simulink model "IEEE33BusTestSystem_Instantaneous"  (R2019a)
settings: Solver=FixedStepAuto  StartTime=0.0  StopTime=0.2  FixedStep=50e-6  RelTol=1e-3
libraries: powerlib x141, powerlib_meascontrol x2
(part 3 of 3)

== system IEEE33BusTestSystem_Instantaneous/Bus_7 ==
  Bus Load 7 : powerlib/Elements/Three-Phase Series RLC Load  LConnTagsString=A|B|C  Configuration=Y (grounded)  NominalVoltage=(12660)*0.946243  Vabc=[1e3 1e3 1e3]  Vabcp=[1e3 1e3 1e3]  NominalFrequency=50  UnbalancedPower=off  ActivePower=200e3  InductivePower=100e3  CapacitivePower=0  Pabc=[10e3 9e3 11e3]  QLabc=[100 90 110]  QCabc=[100 90 110]  Pabcp=[10e3 9e3 11e3]  QLabcp=[100 90 110]  QCabcp=[100 90 110]  Measurements=None  LoadType=constant PQ
      settings: SourceProductName=Simscape Electrical
  Bus_7 : powerlib/Measurements/Three-Phase V-I Measurement  VoltageMeasurement=phase-to-phase  SetLabelV=off  LabelV=Vabc  Vpu=off  VpuLL=off  CurrentMeasurement=yes  SetLabelI=off  LabelI=Iabc  Ipu=off  Pbase=100e6  Vbase=500e3  OutputType=Complex  PhasorSimulation=off  PSBequivalent=0
      settings: SourceProductName=Simscape Electrical
  CB3-2 : powerlib/Elements/Three-Phase Breaker  InitialState=open  SwitchA=on  SwitchB=on  SwitchC=on  SwitchTimes="[1/60  5/60]"  External=on  BreakerResistance=0.01  SnubberResistance=1e6  SnubberCapacitance=inf  Measurements=None
      settings: SourceProductName=Simscape Electrical
  VI Recorder10 : Subsystem
  InPhaseA : PMIOPort  Side=Left
  InPhaseB : PMIOPort  Port=2  Side=Left
  InPhaseC : PMIOPort  Port=3  Side=Left
  OutPhaseA : PMIOPort  Port=4  Side=Right
  OutPhaseB : PMIOPort  Port=5  Side=Right
  OutPhaseC : PMIOPort  Port=6  Side=Right
  wires:
  Bus_7/2 -> VI Recorder10/2(Irec)
  Bus_7/1 -> VI Recorder10/1(Vrec)
  [CB7to8] -> CB3-2/1
  connections:
  Bus_7/RConn1 -- CB3-2/LConn1 -- Bus Load 7/LConn1
  CB3-2/RConn3 -- OutPhaseC/RConn1
  Bus Load 7/LConn2 -- CB3-2/LConn2 -- Bus_7/RConn2
  CB3-2/LConn3 -- Bus Load 7/LConn3 -- Bus_7/RConn3
  CB3-2/RConn1 -- OutPhaseA/RConn1
  CB3-2/RConn2 -- OutPhaseB/RConn1
  InPhaseA/RConn1 -- Bus_7/LConn1
  InPhaseB/RConn1 -- Bus_7/LConn2
  InPhaseC/RConn1 -- Bus_7/LConn3

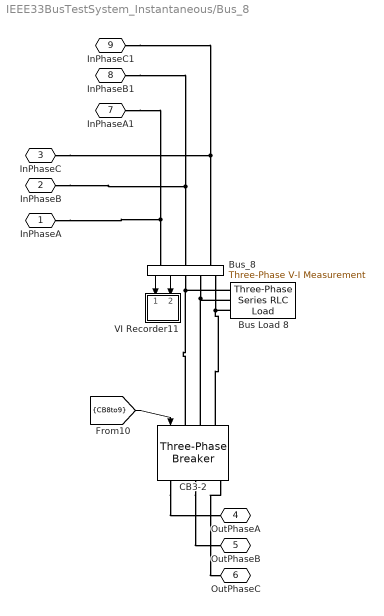
== system IEEE33BusTestSystem_Instantaneous/Bus_8 ==
  Bus Load 8 : powerlib/Elements/Three-Phase Series RLC Load  LConnTagsString=A|B|C  Configuration=Y (grounded)  NominalVoltage=(12660)*0.941407  Vabc=[1e3 1e3 1e3]  Vabcp=[1e3 1e3 1e3]  NominalFrequency=50  UnbalancedPower=off  ActivePower=200e3  InductivePower=100e3  CapacitivePower=0  Pabc=[10e3 9e3 11e3]  QLabc=[100 90 110]  QCabc=[100 90 110]  Pabcp=[10e3 9e3 11e3]  QLabcp=[100 90 110]  QCabcp=[100 90 110]  Measurements=None  LoadType=constant PQ
      settings: SourceProductName=Simscape Electrical
  Bus_8 : powerlib/Measurements/Three-Phase V-I Measurement  VoltageMeasurement=phase-to-phase  SetLabelV=off  LabelV=Vabc  Vpu=off  VpuLL=off  CurrentMeasurement=yes  SetLabelI=off  LabelI=Iabc  Ipu=off  Pbase=100e6  Vbase=500e3  OutputType=Complex  PhasorSimulation=off  PSBequivalent=0
      settings: SourceProductName=Simscape Electrical
  CB3-2 : powerlib/Elements/Three-Phase Breaker  InitialState=open  SwitchA=on  SwitchB=on  SwitchC=on  SwitchTimes="[1/60  5/60]"  External=on  BreakerResistance=0.01  SnubberResistance=1e6  SnubberCapacitance=inf  Measurements=None
      settings: SourceProductName=Simscape Electrical
  VI Recorder11 : Subsystem
  InPhaseA : PMIOPort  Side=Left
  InPhaseB : PMIOPort  Port=2  Side=Left
  InPhaseC : PMIOPort  Port=3  Side=Left
  OutPhaseA : PMIOPort  Port=4  Side=Right
  OutPhaseB : PMIOPort  Port=5  Side=Right
  OutPhaseC : PMIOPort  Port=6  Side=Right
  InPhaseA1 : PMIOPort  Port=7  Side=Left
  InPhaseB1 : PMIOPort  Port=8  Side=Left
  InPhaseC1 : PMIOPort  Port=9  Side=Left
  wires:
  Bus_8/2 -> VI Recorder11/2(Irec)
  Bus_8/1 -> VI Recorder11/1(Vrec)
  [CB8to9] -> CB3-2/1
  connections:
  Bus Load 8/LConn1 -- CB3-2/LConn1 -- Bus_8/RConn1
  CB3-2/RConn3 -- OutPhaseC/RConn1
  Bus Load 8/LConn2 -- CB3-2/LConn2 -- Bus_8/RConn2
  Bus_8/RConn3 -- CB3-2/LConn3 -- Bus Load 8/LConn3
  CB3-2/RConn1 -- OutPhaseA/RConn1
  CB3-2/RConn2 -- OutPhaseB/RConn1
  InPhaseA1/RConn1 -- InPhaseA/RConn1 -- Bus_8/LConn1
  InPhaseB1/RConn1 -- InPhaseB/RConn1 -- Bus_8/LConn2
  InPhaseC1/RConn1 -- InPhaseC/RConn1 -- Bus_8/LConn3

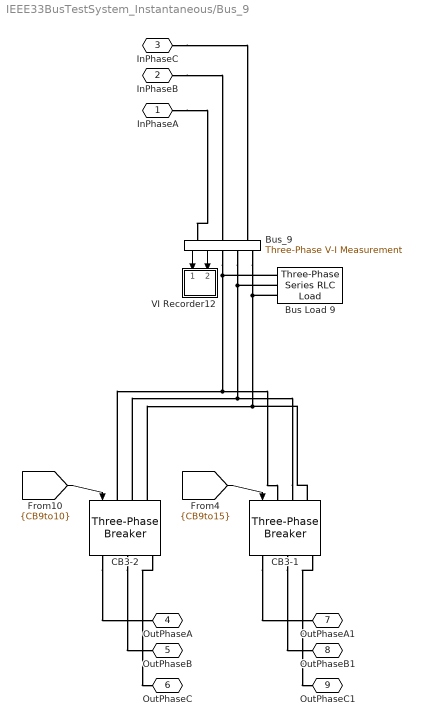
== system IEEE33BusTestSystem_Instantaneous/Bus_9 ==
  Bus Load 9 : powerlib/Elements/Three-Phase Series RLC Load  LConnTagsString=A|B|C  Configuration=Y (grounded)  NominalVoltage=(12660)*0.935148  Vabc=[1e3 1e3 1e3]  Vabcp=[1e3 1e3 1e3]  NominalFrequency=50  UnbalancedPower=off  ActivePower=60e3  InductivePower=20e3  CapacitivePower=0  Pabc=[10e3 9e3 11e3]  QLabc=[100 90 110]  QCabc=[100 90 110]  Pabcp=[10e3 9e3 11e3]  QLabcp=[100 90 110]  QCabcp=[100 90 110]  Measurements=None  LoadType=constant PQ
      settings: SourceProductName=Simscape Electrical
  Bus_9 : powerlib/Measurements/Three-Phase V-I Measurement  VoltageMeasurement=phase-to-phase  SetLabelV=off  LabelV=Vabc  Vpu=off  VpuLL=off  CurrentMeasurement=yes  SetLabelI=off  LabelI=Iabc  Ipu=off  Pbase=100e6  Vbase=500e3  OutputType=Complex  PhasorSimulation=off  PSBequivalent=0
      settings: SourceProductName=Simscape Electrical
  CB3-1 : powerlib/Elements/Three-Phase Breaker  InitialState=open  SwitchA=on  SwitchB=on  SwitchC=on  SwitchTimes="[1/60  5/60]"  External=on  BreakerResistance=0.01  SnubberResistance=1e6  SnubberCapacitance=inf  Measurements=None
      settings: SourceProductName=Simscape Electrical
  CB3-2 : powerlib/Elements/Three-Phase Breaker  InitialState=open  SwitchA=on  SwitchB=on  SwitchC=on  SwitchTimes="[1/60  5/60]"  External=on  BreakerResistance=0.01  SnubberResistance=1e6  SnubberCapacitance=inf  Measurements=None
      settings: SourceProductName=Simscape Electrical
  VI Recorder12 : Subsystem
  InPhaseA : PMIOPort  Side=Left
  InPhaseB : PMIOPort  Port=2  Side=Left
  InPhaseC : PMIOPort  Port=3  Side=Left
  OutPhaseA : PMIOPort  Port=4  Side=Right
  OutPhaseB : PMIOPort  Port=5  Side=Right
  OutPhaseC : PMIOPort  Port=6  Side=Right
  OutPhaseA1 : PMIOPort  Port=7  Side=Right
  OutPhaseB1 : PMIOPort  Port=8  Side=Right
  OutPhaseC1 : PMIOPort  Port=9  Side=Right
  wires:
  Bus_9/2 -> VI Recorder12/2(Irec)
  Bus_9/1 -> VI Recorder12/1(Vrec)
  [CB9to10] -> CB3-2/1
  [CB9to15] -> CB3-1/1
  connections:
  CB3-1/LConn1 -- Bus Load 9/LConn1 -- Bus_9/RConn1 -- CB3-2/LConn1
  CB3-2/RConn3 -- OutPhaseC/RConn1
  CB3-1/LConn2 -- Bus_9/RConn2 -- Bus Load 9/LConn2 -- CB3-2/LConn2
  Bus Load 9/LConn3 -- Bus_9/RConn3 -- CB3-1/LConn3 -- CB3-2/LConn3
  CB3-2/RConn1 -- OutPhaseA/RConn1
  CB3-2/RConn2 -- OutPhaseB/RConn1
  InPhaseA/RConn1 -- Bus_9/LConn1
  InPhaseB/RConn1 -- Bus_9/LConn2
  InPhaseC/RConn1 -- Bus_9/LConn3
  CB3-1/RConn2 -- OutPhaseB1/RConn1
  CB3-1/RConn3 -- OutPhaseC1/RConn1
  CB3-1/RConn1 -- OutPhaseA1/RConn1

== system IEEE33BusTestSystem_Instantaneous/Bus_10/VI Recorder13 ==
  Vrec : Inport
  Irec : Inport  Port=2
  tag scope: I9to10=global, V9to10=global
  wires:
  Vrec/1 -> [V9to10]
  Irec/1 -> [I9to10]

== system IEEE33BusTestSystem_Instantaneous/Bus_11/VI Recorder14 ==
  Vrec : Inport
  Irec : Inport  Port=2
  tag scope: I10to11=global, V10to11=global
  wires:
  Vrec/1 -> [V10to11]
  Irec/1 -> [I10to11]

== system IEEE33BusTestSystem_Instantaneous/Bus_12/VI Recorder15 ==
  Vrec : Inport
  Irec : Inport  Port=2
  tag scope: I11to12=global, V11to12=global
  wires:
  Vrec/1 -> [V11to12]
  Irec/1 -> [I11to12]

== system IEEE33BusTestSystem_Instantaneous/Bus_13/VI Recorder16 ==
  Vrec : Inport
  Irec : Inport  Port=2
  tag scope: I12to13=global, V12to13=global
  wires:
  Vrec/1 -> [V12to13]
  Irec/1 -> [I12to13]

== system IEEE33BusTestSystem_Instantaneous/Bus_14/VI Recorder17 ==
  Vrec : Inport
  Irec : Inport  Port=2
  tag scope: I13to14=global, V13to14=global
  wires:
  Vrec/1 -> [V13to14]
  Irec/1 -> [I13to14]

== system IEEE33BusTestSystem_Instantaneous/Bus_15/VI Recorder18 ==
  Vrec : Inport
  Irec : Inport  Port=2
  tag scope: I14to15=global, V14to15=global
  wires:
  Vrec/1 -> [V14to15]
  Irec/1 -> [I14to15]

== system IEEE33BusTestSystem_Instantaneous/Bus_16/VI Recorder19 ==
  Vrec : Inport
  Irec : Inport  Port=2
  tag scope: I15to16=global, V15to16=global
  wires:
  Vrec/1 -> [V15to16]
  Irec/1 -> [I15to16]

== system IEEE33BusTestSystem_Instantaneous/Bus_17/VI Recorder20 ==
  Vrec : Inport
  Irec : Inport  Port=2
  tag scope: I16to17=global, V16to17=global
  wires:
  Vrec/1 -> [V16to17]
  Irec/1 -> [I16to17]

== system IEEE33BusTestSystem_Instantaneous/Bus_18/VI Recorder21 ==
  Vrec : Inport
  Irec : Inport  Port=2
  tag scope: I17to18=global, V17to18=global
  wires:
  Vrec/1 -> [V17to18]
  Irec/1 -> [I17to18]

== system IEEE33BusTestSystem_Instantaneous/Bus_19/VI Recorder ==
  Vrec : Inport
  Irec : Inport  Port=2
  tag scope: I2to19=global, V2to19=global
  wires:
  Vrec/1 -> [V2to19]
  Irec/1 -> [I2to19]

== system IEEE33BusTestSystem_Instantaneous/Bus_2/VI Recorder5 ==
  Vrec : Inport
  Irec : Inport  Port=2
  tag scope: I1to2=global, V1to2=global
  wires:
  Vrec/1 -> [V1to2]
  Irec/1 -> [I1to2]

== system IEEE33BusTestSystem_Instantaneous/Bus_20/VI Recorder1 ==
  Vrec : Inport
  Irec : Inport  Port=2
  tag scope: I19to20=global, V19to20=global
  wires:
  Vrec/1 -> [V19to20]
  Irec/1 -> [I19to20]

== system IEEE33BusTestSystem_Instantaneous/Bus_21/VI Recorder2 ==
  Vrec : Inport
  Irec : Inport  Port=2
  tag scope: I20to21=global, V20to21=global
  wires:
  Vrec/1 -> [V20to21]
  Irec/1 -> [I20to21]

== system IEEE33BusTestSystem_Instantaneous/Bus_22/VI Recorder3 ==
  Vrec : Inport
  Irec : Inport  Port=2
  tag scope: I21to22=global, V21to22=global
  wires:
  Vrec/1 -> [V21to22]
  Irec/1 -> [I21to22]

== system IEEE33BusTestSystem_Instantaneous/Bus_23/VI Recorder32 ==
  Vrec : Inport
  Irec : Inport  Port=2
  tag scope: I3to23=global, V3to23=global
  wires:
  Vrec/1 -> [V3to23]
  Irec/1 -> [I3to23]

== system IEEE33BusTestSystem_Instantaneous/Bus_24/VI Recorder31 ==
  Vrec : Inport
  Irec : Inport  Port=2
  tag scope: I23to24=global, V23to24=global
  wires:
  Vrec/1 -> [V23to24]
  Irec/1 -> [I23to24]

== system IEEE33BusTestSystem_Instantaneous/Bus_25/VI Recorder30 ==
  Vrec : Inport
  Irec : Inport  Port=2
  tag scope: I24to25=global, V24to25=global
  wires:
  Vrec/1 -> [V24to25]
  Irec/1 -> [I24to25]

== system IEEE33BusTestSystem_Instantaneous/Bus_26/VI Recorder22 ==
  Vrec : Inport
  Irec : Inport  Port=2
  tag scope: I6to26=global, V6to26=global
  wires:
  Vrec/1 -> [V6to26]
  Irec/1 -> [I6to26]

== system IEEE33BusTestSystem_Instantaneous/Bus_27/VI Recorder23 ==
  Vrec : Inport
  Irec : Inport  Port=2
  tag scope: I26to27=global, V26to27=global
  wires:
  Vrec/1 -> [V26to27]
  Irec/1 -> [I26to27]

== system IEEE33BusTestSystem_Instantaneous/Bus_28/VI Recorder24 ==
  Vrec : Inport
  Irec : Inport  Port=2
  tag scope: I27to28=global, V27to28=global
  wires:
  Vrec/1 -> [V27to28]
  Irec/1 -> [I27to28]

== system IEEE33BusTestSystem_Instantaneous/Bus_29/VI Recorder25 ==
  Vrec : Inport
  Irec : Inport  Port=2
  tag scope: I28to29=global, V28to29=global
  wires:
  Vrec/1 -> [V28to29]
  Irec/1 -> [I28to29]

== system IEEE33BusTestSystem_Instantaneous/Bus_3/VI Recorder6 ==
  Vrec : Inport
  Irec : Inport  Port=2
  tag scope: I2to3=global, V2to3=global
  wires:
  Vrec/1 -> [V2to3]
  Irec/1 -> [I2to3]

== system IEEE33BusTestSystem_Instantaneous/Bus_30/VI Recorder26 ==
  Vrec : Inport
  Irec : Inport  Port=2
  tag scope: I29to30=global, V29to30=global
  wires:
  Vrec/1 -> [V29to30]
  Irec/1 -> [I29to30]

== system IEEE33BusTestSystem_Instantaneous/Bus_31/VI Recorder27 ==
  Vrec : Inport
  Irec : Inport  Port=2
  tag scope: I30to31=global, V30to31=global
  wires:
  Vrec/1 -> [V30to31]
  Irec/1 -> [I30to31]

== system IEEE33BusTestSystem_Instantaneous/Bus_32/VI Recorder28 ==
  Vrec : Inport
  Irec : Inport  Port=2
  tag scope: I31to32=global, V31to32=global
  wires:
  Vrec/1 -> [V31to32]
  Irec/1 -> [I31to32]

== system IEEE33BusTestSystem_Instantaneous/Bus_33/VI Recorder29 ==
  Vrec : Inport
  Irec : Inport  Port=2
  tag scope: I32to33=global, V32to33=global
  wires:
  Vrec/1 -> [V32to33]
  Irec/1 -> [I32to33]

== system IEEE33BusTestSystem_Instantaneous/Bus_4/VI Recorder7 ==
  Vrec : Inport
  Irec : Inport  Port=2
  tag scope: I3to4=global, V3to4=global
  wires:
  Vrec/1 -> [V3to4]
  Irec/1 -> [I3to4]

== system IEEE33BusTestSystem_Instantaneous/Bus_5/VI Recorder8 ==
  Vrec : Inport
  Irec : Inport  Port=2
  tag scope: I4to5=global, V4to5=global
  wires:
  Vrec/1 -> [V4to5]
  Irec/1 -> [I4to5]

== system IEEE33BusTestSystem_Instantaneous/Bus_6/VI Recorder9 ==
  Vrec : Inport
  Irec : Inport  Port=2
  tag scope: I5to6=global, V5to6=global
  wires:
  Vrec/1 -> [V5to6]
  Irec/1 -> [I5to6]

== system IEEE33BusTestSystem_Instantaneous/Bus_7/VI Recorder10 ==
  Vrec : Inport
  Irec : Inport  Port=2
  tag scope: I6to7=global, V6to7=global
  wires:
  Vrec/1 -> [V6to7]
  Irec/1 -> [I6to7]

== system IEEE33BusTestSystem_Instantaneous/Bus_8/VI Recorder11 ==
  Vrec : Inport
  Irec : Inport  Port=2
  tag scope: I7to8=global, V7to8=global
  wires:
  Vrec/1 -> [V7to8]
  Irec/1 -> [I7to8]

== system IEEE33BusTestSystem_Instantaneous/Bus_9/VI Recorder12 ==
  Vrec : Inport
  Irec : Inport  Port=2
  tag scope: I8to9=global, V8to9=global
  wires:
  Vrec/1 -> [V8to9]
  Irec/1 -> [I8to9]
